simulink model "Thermostat_Control"  (R2024b)
settings: Solver=VariableStepAuto  StartTime=0.0  StopTime=120  RelTol=1e-3
settings Model: Creator=HP  LastModifiedBy=HP

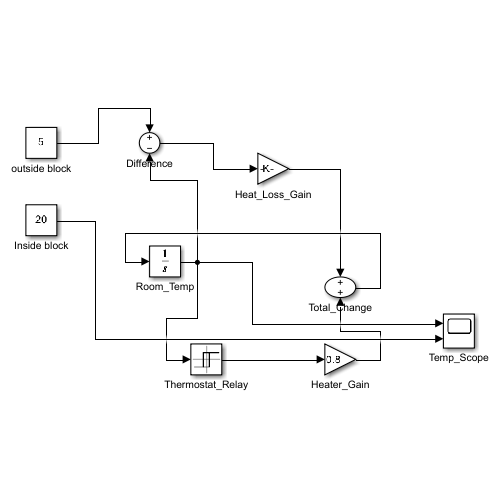
[thumbnail: Simulink's stored preview of the top-level diagram]
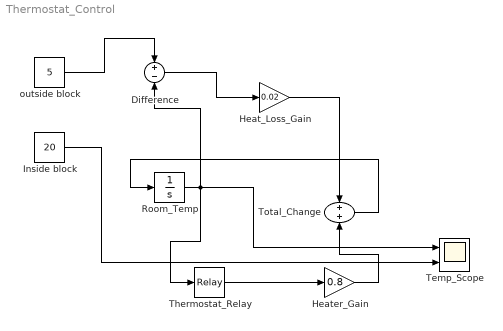
== system Thermostat_Control ==
  Difference : Sum  Inputs=+-
  Heat_Loss_Gain : Gain  Gain=0.02
  Heater_Gain : Gain  Gain=0.8
  Inside block : Constant  Value=20
  Room_Temp : Integrator  InitialCondition=15
  Temp_Scope : Scope  NumInputPorts=2
  Thermostat_Relay : Relay  OnSwitchValue=21  OffSwitchValue=19  OnOutputValue=0  OffOutputValue=1
  Total_Change : Sum
  outside block : Constant  Value=5
  wires:
  outside block/1 -> Difference/1
  Room_Temp/1 -> Temp_Scope/1, Difference/2, Thermostat_Relay/1
  Thermostat_Relay/1 -> Heater_Gain/1
  Heater_Gain/1 -> Total_Change/2
  Heat_Loss_Gain/1 -> Total_Change/1
  Difference/1 -> Heat_Loss_Gain/1
  Inside block/1 -> Temp_Scope/2
  Total_Change/1 -> Room_Temp/1
